simulink model "sps_device_closed_loop"  (R2023b)
settings: Solver=FixedStepDiscrete  StartTime=0.0  StopTime=0.23999999999999999  FixedStep=1.2499999999999999e-07  RelTol=1e-3
libraries: spsCurrentMeasurementLib x4, spsMosfetLib x4, spsSeriesRLCBranchLib x3, spsVoltageMeasurementLib x2, spsGroundLib x1, spsDCVoltageSourceLib x1, sps_lib x1
Description:
  | Device stage: four explicit Specialized Power Systems MOSFET blocks with antiparallel body diodes, physical DC source and LC/load network.
settings Model: Creator=Oll1ver  LastModifiedBy=Oll1ver
settings DataIOCC: SaveOutput=off  SaveTime=off

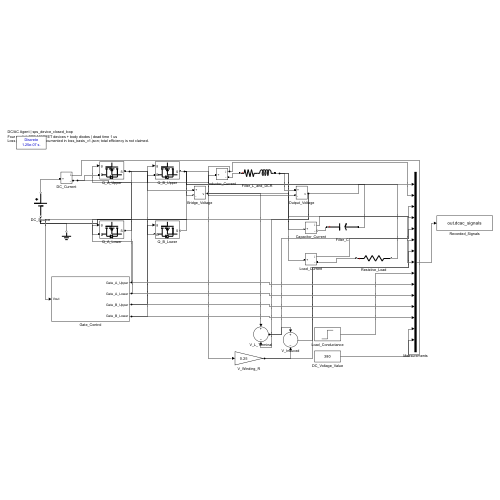
[thumbnail: Simulink's stored preview of the top-level diagram]
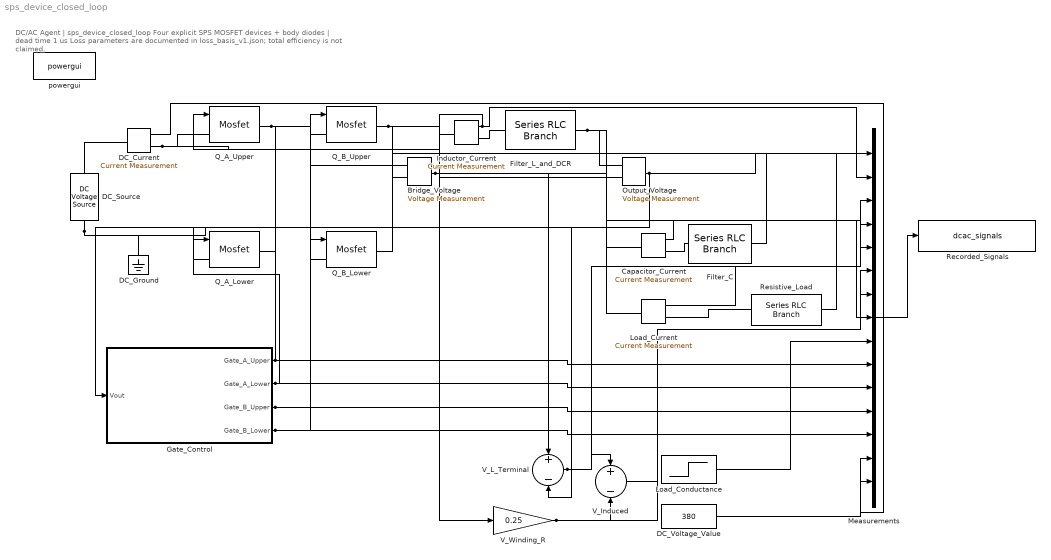
== system sps_device_closed_loop ==
  note: DC/AC Agent | sps_device_closed_loop
      | Four explicit SPS MOSFET devices + body diodes | dead time 1 us
      | Loss parameters are documented in loss_basis_v1.json; total efficiency is not claimed.
  Bridge_Voltage : spsVoltageMeasurementLib/Voltage Measurement  PhasorSimulation=off  OutputType=Complex  PSBequivalent=0
  Capacitor_Current : spsCurrentMeasurementLib/Current Measurement  PhasorSimulation=off  OutputType=Complex  PSBequivalent=0
  DC_Current : spsCurrentMeasurementLib/Current Measurement  PhasorSimulation=off  OutputType=Complex  PSBequivalent=0
  DC_Ground : spsGroundLib/Ground  LConnTagsString=a
  DC_Source : spsDCVoltageSourceLib/DC Voltage Source  Amplitude=380  Measurements=None
  DC_Voltage_Value : Constant  Value=380
  Filter_C : spsSeriesRLCBranchLib/Series RLC Branch  LConnTagsString=__new0  RConnTagsString=__new0  BranchType=C  Resistance=1  Inductance=1e-3  SetiL0=off  InitialCurrent=0  Capacitance=4.6999999999999999e-06  Setx0=off  InitialVoltage=0  Measurements=None
  Filter_L_and_DCR : spsSeriesRLCBranchLib/Series RLC Branch  LConnTagsString=__new0  RConnTagsString=__new0  BranchType=RL  Resistance=0.25  Inductance=0.002  SetiL0=off  InitialCurrent=0  Capacitance=1e-6  Setx0=off  InitialVoltage=0  Measurements=None
  Gate_Control : Subsystem
  Inductor_Current : spsCurrentMeasurementLib/Current Measurement  PhasorSimulation=off  OutputType=Complex  PSBequivalent=0
  Load_Conductance : Step  Time=0.12  Before=0.010330578512396695  After=0.010330578512396695  SampleTime=0
  Load_Current : spsCurrentMeasurementLib/Current Measurement  PhasorSimulation=off  OutputType=Complex  PSBequivalent=0
  Measurements : Mux  Inputs=15
  Output_Voltage : spsVoltageMeasurementLib/Voltage Measurement  PhasorSimulation=off  OutputType=Complex  PSBequivalent=0
  Q_A_Lower : spsMosfetLib/Mosfet  Ron=0.075999999999999998  Lon=0  Rd=0.001  Vfd=1  IC=0  Rs=1e6  Cs=inf  Measurements=off
  Q_A_Upper : spsMosfetLib/Mosfet  Ron=0.075999999999999998  Lon=0  Rd=0.001  Vfd=1  IC=0  Rs=1e6  Cs=inf  Measurements=off
  Q_B_Lower : spsMosfetLib/Mosfet  Ron=0.075999999999999998  Lon=0  Rd=0.001  Vfd=1  IC=0  Rs=1e6  Cs=inf  Measurements=off
  Q_B_Upper : spsMosfetLib/Mosfet  Ron=0.075999999999999998  Lon=0  Rd=0.001  Vfd=1  IC=0  Rs=1e6  Cs=inf  Measurements=off
  Recorded_Signals : ToWorkspace  VariableName=dcac_signals  SaveFormat=Timeseries  SampleTime=-1
  Resistive_Load : spsSeriesRLCBranchLib/Series RLC Branch  LConnTagsString=__new0  RConnTagsString=__new0  BranchType=R  Resistance=96.799999999999997  Inductance=1e-3  SetiL0=off  InitialCurrent=0  Capacitance=1e-6  Setx0=off  InitialVoltage=0  Measurements=None
  V_Induced : Sum  Inputs=+-
  V_L_Terminal : Sum  Inputs=+-
  V_Winding_R : Gain  Gain=0.25
  powergui : sps_lib/powergui  Priority=1  SimulationMode=Discrete  SampleTime=1.2499999999999999e-07  frequency=50  Iterations=50  frequencyindice=0  Pbase=100e6  ErrMax=1e-4  UnitsV=kV  UnitsW=MW  buscounter=0  FunctionMessages=off  echomessages=off  EnableUseOfTLC=off  CurrentSourceSwitches=off  DisableSnubberDevices=off  DisableRonSwitches=off  DisableVfSwitches=off  DisplayEquations=off  AutomaticDiscreteSolvers=off  SolverType=Tustin/Backward Euler (TBE)  Interpol=off  ExternalGateDelay=off  methode=off  Ts=100  x0status=blocks  SPID=on  SwTol=0  HookPort=off  NonlinearTolerance=1e-4  nMaxIteration=100  ContinueOnMaxIteration=off  RestoreLinks=warning  ResistiveCurrentMeasurement=off  Frange=[0:2:500]  Ylog=off  Xlog=on  ShowGrid=off  save=off  variable=ZData  structure=0  ZoomFFT=off  StartTime=0.0  cycles=1  DisplayStyle=1  fundamental=60  FreqAxis=off  MaxFrequency=1000  frequencyindicesteady=1  RmsSteady=1  display=off
  wires:
  Gate_Control/1(Gate_A_Upper) -> Q_A_Upper/1, Measurements/10
  Gate_Control/2(Gate_A_Lower) -> Q_A_Lower/1, Measurements/11
  Gate_Control/3(Gate_B_Upper) -> Q_B_Upper/1, Measurements/12
  Gate_Control/4(Gate_B_Lower) -> Q_B_Lower/1, Measurements/13
  Output_Voltage/1 -> Gate_Control/1(Vout), V_L_Terminal/2, Measurements/1
  Bridge_Voltage/1 -> V_L_Terminal/1, Measurements/4
  Inductor_Current/1 -> V_Winding_R/1, Measurements/2
  V_L_Terminal/1 -> V_Induced/1, Measurements/5
  V_Winding_R/1 -> V_Induced/2, Measurements/6
  Load_Current/1 -> Measurements/3
  V_Induced/1 -> Measurements/7
  Capacitor_Current/1 -> Measurements/8
  Load_Conductance/1 -> Measurements/9
  DC_Current/1 -> Measurements/14
  DC_Voltage_Value/1 -> Measurements/15
  Measurements/1 -> Recorded_Signals/1
  connections:
  DC_Source/RConn1 -- DC_Current/LConn1
  Q_A_Upper/LConn1 -- DC_Current/RConn1 -- Q_B_Upper/LConn1
  Q_A_Lower/RConn1 -- DC_Source/LConn1 -- Q_B_Lower/RConn1 -- DC_Ground/LConn1
  Q_A_Lower/LConn1 -- Q_A_Upper/RConn1 -- Inductor_Current/LConn1 -- Bridge_Voltage/LConn1
  Q_B_Lower/LConn1 -- Q_B_Upper/RConn1 -- Bridge_Voltage/LConn2 -- Output_Voltage/LConn2 -- Filter_C/RConn1 -- Resistive_Load/RConn1
  Inductor_Current/RConn1 -- Filter_L_and_DCR/LConn1
  Output_Voltage/LConn1 -- Filter_L_and_DCR/RConn1 -- Capacitor_Current/LConn1 -- Load_Current/LConn1
  Capacitor_Current/RConn1 -- Filter_C/LConn1
  Load_Current/RConn1 -- Resistive_Load/LConn1

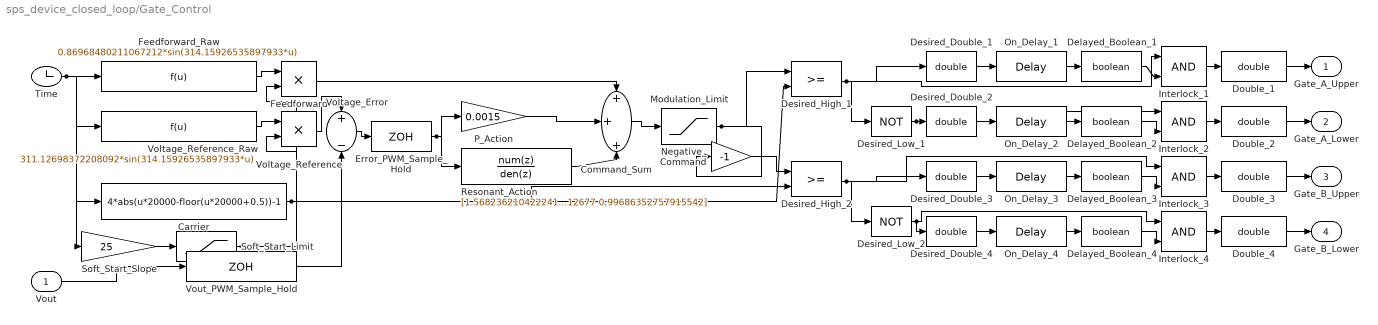
== system sps_device_closed_loop/Gate_Control ==
  Vout : Inport
  Carrier : Fcn  Expr=4*abs(u*20000-floor(u*20000+0.5))-1
  Command_Sum : Sum  Inputs=+++
  Delayed_Boolean_{1..4} (4 alike) : DataTypeConversion  OutDataTypeStr=boolean  SaturateOnIntegerOverflow=off  RndMeth=Floor
  Desired_Double_{1..4} (4 alike) : DataTypeConversion  OutDataTypeStr=double  SaturateOnIntegerOverflow=off  RndMeth=Floor
  Desired_High_1 : RelationalOperator  OutDataTypeStr=boolean  RndMeth=Simplest  InputSameDT=off
  Desired_High_2 : RelationalOperator  OutDataTypeStr=boolean  RndMeth=Simplest  InputSameDT=off
  Desired_Low_1 : Logic  Operator=NOT  AllPortsSameDT=off  OutDataTypeStr=boolean
  Desired_Low_2 : Logic  Operator=NOT  AllPortsSameDT=off  OutDataTypeStr=boolean
  Double_{1..4} (4 alike) : DataTypeConversion  OutDataTypeStr=double  SaturateOnIntegerOverflow=off  RndMeth=Floor
  Error_PWM_Sample_Hold : ZeroOrderHold  SampleTime=5.0000000000000002e-05
  Feedforward : Product
  Feedforward_Raw : Fcn  Expr=0.86968480211067212*sin(314.15926535897933*u)
  Interlock_{1..4} (4 alike) : Logic  AllPortsSameDT=off  OutDataTypeStr=boolean
  Modulation_Limit : Saturate  UpperLimit=0.94999999999999996  LowerLimit=-0.94999999999999996
  Negative_Command : Gain  Gain=-1
  On_Delay_{1..4} (4 alike) : TransportDelay  DelayTime=9.9999999999999995e-07
  P_Action : Gain  Gain=0.0015
  Resonant_Action : DiscreteTransferFcn  Numerator=[1.5682362104222414e-05 0 -1.5682362104222414e-05]  Denominator=[1 -1.9966171896112677 0.99686352757915542]  SampleTime=5.0000000000000002e-05
  Soft_Start_Limit : Saturate  UpperLimit=1  LowerLimit=0
  Soft_Start_Slope : Gain  Gain=25
  Time : Clock
  Voltage_Error : Sum  Inputs=+-
  Voltage_Reference : Product
  Voltage_Reference_Raw : Fcn  Expr=311.12698372208092*sin(314.15926535897933*u)
  Vout_PWM_Sample_Hold : ZeroOrderHold  SampleTime=5.0000000000000002e-05
  Gate_A_Upper : Outport
  Gate_A_Lower : Outport  Port=2
  Gate_B_Upper : Outport  Port=3
  Gate_B_Lower : Outport  Port=4
  wires:
  Time/1 -> Carrier/1, Soft_Start_Slope/1, Feedforward_Raw/1, Voltage_Reference_Raw/1
  Soft_Start_Slope/1 -> Soft_Start_Limit/1
  Feedforward_Raw/1 -> Feedforward/1
  Soft_Start_Limit/1 -> Feedforward/2, Voltage_Reference/2
  Voltage_Reference_Raw/1 -> Voltage_Reference/1
  Voltage_Reference/1 -> Voltage_Error/1
  Vout/1 -> Vout_PWM_Sample_Hold/1
  Vout_PWM_Sample_Hold/1 -> Voltage_Error/2
  Voltage_Error/1 -> Error_PWM_Sample_Hold/1
  Error_PWM_Sample_Hold/1 -> P_Action/1, Resonant_Action/1
  Feedforward/1 -> Command_Sum/1
  P_Action/1 -> Command_Sum/2
  Resonant_Action/1 -> Command_Sum/3
  Command_Sum/1 -> Modulation_Limit/1
  Modulation_Limit/1 -> Negative_Command/1, Desired_High_1/1
  Carrier/1 -> Desired_High_1/2, Desired_High_2/2
  Desired_High_1/1 -> Desired_Low_1/1, Desired_Double_1/1, Interlock_1/1
  Negative_Command/1 -> Desired_High_2/1
  Desired_High_2/1 -> Desired_Low_2/1, Desired_Double_3/1, Interlock_3/1
  Desired_Double_1/1 -> On_Delay_1/1
  On_Delay_1/1 -> Delayed_Boolean_1/1
  Delayed_Boolean_1/1 -> Interlock_1/2
  Interlock_1/1 -> Double_1/1
  Double_1/1 -> Gate_A_Upper/1
  Desired_Low_1/1 -> Desired_Double_2/1, Interlock_2/1
  Desired_Double_2/1 -> On_Delay_2/1
  On_Delay_2/1 -> Delayed_Boolean_2/1
  Delayed_Boolean_2/1 -> Interlock_2/2
  Interlock_2/1 -> Double_2/1
  Double_2/1 -> Gate_A_Lower/1
  Desired_Double_3/1 -> On_Delay_3/1
  On_Delay_3/1 -> Delayed_Boolean_3/1
  Delayed_Boolean_3/1 -> Interlock_3/2
  Interlock_3/1 -> Double_3/1
  Double_3/1 -> Gate_B_Upper/1
  Desired_Low_2/1 -> Desired_Double_4/1, Interlock_4/1
  Desired_Double_4/1 -> On_Delay_4/1
  On_Delay_4/1 -> Delayed_Boolean_4/1
  Delayed_Boolean_4/1 -> Interlock_4/2
  Interlock_4/1 -> Double_4/1
  Double_4/1 -> Gate_B_Lower/1
